simulink model "afe_rst_inv_psm_distributed_control_two_delays"  (R2026a)
settings: Solver=ode1be  StopTime=simlength  FixedStep=tc  MaxStep=Tc
values from neighbouring files (symbols this model uses):
  Amplitude_U = 1.16    [grid_fault_generator.m]
  Amplitude_V = Amplitude_U    (= 1.16)    [grid_fault_generator.m]
  Amplitude_W = Amplitude_U    (= 1.16)    [grid_fault_generator.m]
  end_time_LVRT = start_time_LVRT + error_length    [grid_fault_generator.m]
  Igrid_phase_normalization_factor = 270*sqrt(2)    [grid_emulator.m]
  omega_grid_emulator_nom = w_grid    (= 314.159265359)    [grid_emulator.m]
  omega_grid_nom = w_grid    (= 314.159265359)    [grid_emulator.m]
  t_ramp = 20e-3    (= 0.02)    [grid_fault_generator.m]
  ugrid_factor = 1    [grid_emulator.m]
  V_phase_normalization_factor = Vgrid_phase_normalization_factor    [grid_emulator.m]
  Vdc_bez = 1070    [grid_emulator.m]
  Vemu_ref_norm = Vemu_ref * sqrt(2) / V_phase_normalization_factor    [grid_emulator.m]
  vn_eta_pu = 0    [grid_emulator.m]
  vn_xi_pu = 0    [grid_emulator.m]
  vp_xi_pu = 1    [grid_emulator.m]
undefined symbols (not defined in the file or in its folder): Adrso, Aresd, Bresd, CFi, CFu, Cresd, Crso, CTRPIFF_CLIP_RELEASE, dead_time_INV, emf_fb_p, emf_fb_p_ccaller_1, emf_fb_p_ccaller_2, emf_p, emf_p_ccaller_1, emf_p_ccaller_2, fPWM_INV, g0_161Hz, g0_500Hz, g1_161Hz, g1_500Hz, i_grid_neg_eta_lim, i_grid_neg_eta_red_lim, i_grid_neg_xi_lim, i_grid_neg_xi_red_lim, i_grid_pos_eta_lim, i_grid_pos_eta_red_lim, ibez, id_lim, ieta_neg_ref_lim, ieta_pos_ref_lim, iq_lim, ixi_pos_ref_lim, Jm_norm, k_frt_ref, kg, ki_afe, ki_i, ki_id, ki_iq, ki_rc_neg_grid, ki_rc_pos_grid, ki_vs, ki_w, kp_afe, kp_i, kp_id, kp_iq, kp_rc_neg_grid, kp_rc_pos_grid, kp_vs, kp_w, kw, l1, l2, Lalpha_norm, Ld_norm, Ldrso, Lq_norm, Ls_norm, luenberger_l1 ... (+30)
libraries: fl_lib x146, nesl_utility x62, simulink x8, cstblocks_lti x7, sl_discontinuities x3, single_phase_transformer_lib x3, flexshaft_lib x1, permanent_magnet_synchronous_machine x1
(part 6 of 14)

== system afe_rst_inv_psm_distributed_control_two_delays/AFE-Modular/afe_leg_b/modulator/sv_pwm ==
  ab : Inport
  enable : Inport  Port=2
  Bus Selector : BusSelector  OutputSignals=da,db,dc
  Bus Selector1 : BusSelector  OutputSignals=us_alpha_ctrl,us_beta_ctrl
  C Caller : CCaller  FunctionName=sv_pwm_process_simulink  PortSpecificationStruct="%)30     .    N @   8    (     @         %    \"     4    !     0         %  0 \"0    $    _    07)G3F%M90  4&]R=$YA;64 4V-O<&4     26YD97@     5'EP90      4VEZ90      27-';&]B86P   X    P    !@    @    $          4    (     0    ,    !         !   P!O=70 #@   #     &    \"     0         !0    @    !     P    $         $  # &]U=  .    .     8    (    !          %    \"     $    &     0         0   ...(+2630 chars)"  SampleTime=ts_afe
  Constant : Constant  Value=ts_afe
  Data Type Conversion1 : DataTypeConversion  OutDataTypeStr=double  SaturateOnIntegerOverflow=off  RndMeth=Floor
  Data Type Conversion15 : DataTypeConversion  OutDataTypeStr=single  SaturateOnIntegerOverflow=off  RndMeth=Floor
  Data Type Conversion16 : DataTypeConversion  OutDataTypeStr=single  SaturateOnIntegerOverflow=off  RndMeth=Floor
  Data Type Conversion17 : DataTypeConversion  OutDataTypeStr=uint32  SaturateOnIntegerOverflow=off  RndMeth=Floor
  Data Type Conversion18 : DataTypeConversion  OutDataTypeStr=single  SaturateOnIntegerOverflow=off  RndMeth=Floor
  Data Type Conversion2 : DataTypeConversion  OutDataTypeStr=double  SaturateOnIntegerOverflow=off  RndMeth=Floor
  Data Type Conversion3 : DataTypeConversion  OutDataTypeStr=double  SaturateOnIntegerOverflow=off  RndMeth=Floor
  Zero-Order Hold{,1..3} (4 alike) : ZeroOrderHold  SampleTime=ts_afe
  modulator : Subsystem
  firing_gates : Outport
  wires:
  Bus Selector/3 -> Data Type Conversion3/1  "<dc>"
  Bus Selector/2 -> Data Type Conversion2/1  "<db>"
  Bus Selector/1 -> Data Type Conversion1/1  "<da>"
  Data Type Conversion1/1 -> modulator/1(u)  "du"
  Data Type Conversion2/1 -> modulator/2(v)  "dv"
  Data Type Conversion3/1 -> modulator/3(w)  "dw"
  Bus Selector1/2 -> Data Type Conversion15/1  "<us_beta_ctrl>"
  Bus Selector1/1 -> Data Type Conversion18/1  "<us_alpha_ctrl>"
  ab/1 -> Bus Selector1/1
  modulator/1(firing_gates) -> firing_gates/1
  C Caller/1 -> Bus Selector/1  "out"
  Data Type Conversion15/1 -> Zero-Order Hold1/1
  Zero-Order Hold3/1 -> C Caller/4
  Data Type Conversion17/1 -> Zero-Order Hold3/1
  Zero-Order Hold1/1 -> C Caller/2
  Data Type Conversion16/1 -> Zero-Order Hold2/1
  enable/1 -> Data Type Conversion17/1
  Data Type Conversion18/1 -> Zero-Order Hold/1
  Constant/1 -> Data Type Conversion16/1
  Zero-Order Hold2/1 -> C Caller/3
  Zero-Order Hold/1 -> C Caller/1

== system afe_rst_inv_psm_distributed_control_two_delays/AFE-Modular/afe_leg_b/solid_state_inverter/switch_1 ==
  Diode : fl_lib/Electrical/Electrical Elements/Diode  Vf=Vgamma V  Ron=Ron Ohm  Goff=1e-8 1/Ohm  i_specify=off  i_priority=None  i=0 A  i_nominal_specify=off  i_nominal_value=1  i_nominal_unit=A  v_specify=off  v_priority=None  v=0 V  v_nominal_specify=off  v_nominal_value=1  v_nominal_unit=V
  Switch : fl_lib/Electrical/Electrical Elements/Switch  R_closed=Ron Ohm  G_open=1e-8 1/Ohm  Threshold=7.5  i_specify=off  i_priority=None  i=0 A  i_nominal_specify=off  i_nominal_value=1  i_nominal_unit=A  v_specify=off  v_priority=None  v=0 V  v_nominal_specify=off  v_nominal_value=1  v_nominal_unit=V
  snubber : fl_lib/Electrical/Electrical Elements/Capacitor  c=Csnubber F  r=Rsnubber Ohm  g=0 1/Ohm  i_specify=off  i_priority=None  i=0 A  i_nominal_specify=off  i_nominal_value=1  i_nominal_unit=A  v_specify=off  v_priority=None  v=0 V  v_nominal_specify=off  v_nominal_value=1  v_nominal_unit=V  vc_specify=off  vc_priority=High  vc=0 V  vc_nominal_specify=off  vc_nominal_value=1  vc_nominal_unit=V
  G : PMIOPort  Side=Left
  C : PMIOPort  Port=2  Side=Left
  E : PMIOPort  Port=3  Side=Right
  connections:
  Diode/LConn1 -- snubber/RConn1 -- E/RConn1 -- Switch/LConn1
  Switch/RConn1 -- G/RConn1
  Diode/RConn1 -- snubber/LConn1 -- C/RConn1 -- Switch/RConn2

== system afe_rst_inv_psm_distributed_control_two_delays/AFE-Modular/afe_leg_b/solid_state_inverter/switch_2 ==
  Diode : fl_lib/Electrical/Electrical Elements/Diode  Vf=Vgamma V  Ron=Ron Ohm  Goff=1e-8 1/Ohm  i_specify=off  i_priority=None  i=0 A  i_nominal_specify=off  i_nominal_value=1  i_nominal_unit=A  v_specify=off  v_priority=None  v=0 V  v_nominal_specify=off  v_nominal_value=1  v_nominal_unit=V
  Switch : fl_lib/Electrical/Electrical Elements/Switch  R_closed=Ron Ohm  G_open=1e-8 1/Ohm  Threshold=7.5  i_specify=off  i_priority=None  i=0 A  i_nominal_specify=off  i_nominal_value=1  i_nominal_unit=A  v_specify=off  v_priority=None  v=0 V  v_nominal_specify=off  v_nominal_value=1  v_nominal_unit=V
  snubber : fl_lib/Electrical/Electrical Elements/Capacitor  c=Csnubber F  r=Rsnubber Ohm  g=0 1/Ohm  i_specify=off  i_priority=None  i=0 A  i_nominal_specify=off  i_nominal_value=1  i_nominal_unit=A  v_specify=off  v_priority=None  v=0 V  v_nominal_specify=off  v_nominal_value=1  v_nominal_unit=V  vc_specify=off  vc_priority=High  vc=0 V  vc_nominal_specify=off  vc_nominal_value=1  vc_nominal_unit=V
  G : PMIOPort  Side=Left
  C : PMIOPort  Port=2  Side=Left
  E : PMIOPort  Port=3  Side=Right
  connections:
  Diode/RConn1 -- snubber/LConn1 -- Switch/RConn2 -- C/RConn1
  Switch/RConn1 -- G/RConn1
  Diode/LConn1 -- snubber/RConn1 -- Switch/LConn1 -- E/RConn1

== system afe_rst_inv_psm_distributed_control_two_delays/AFE-Modular/afe_leg_c/driver_board_c/current_ctrl ==
  i_xi_ref : Inport
  phase_current_control : Subsystem
  xieta2abc : Subsystem
  us_alphabeta_ctrl : Outport
  wires:
  i_xi_ref/1 -> xieta2abc/1(pos_xi)  "i_xi_ref"
  phase_current_control/1(us_alphabeta_ctrl) -> us_alphabeta_ctrl/1
  xieta2abc/1(i_abc_reference) -> phase_current_control/1(In1)
  [gamma_grid_dbc] -> xieta2abc/5(gamma)
  [isc_pu_dbc] -> phase_current_control/2(is_abc)
  [is_eta_pos_ref_mb_fb_dbc] -> xieta2abc/2(pos_eta)
  [is_xi_neg_ref_mb_fb_dbc] -> xieta2abc/3(neg_xi)
  [is_eta_neg_ref_mb_fb_dbc] -> xieta2abc/4(neg_eta)

== system afe_rst_inv_psm_distributed_control_two_delays/AFE-Modular/afe_leg_c/driver_board_c/dq_pll ==
  pll_stageA : Subsystem
  pll_stageB : Subsystem
  tag scope: gamma_grid_dbc=global
  wires:
  pll_stageB/1(gamma_grid_pll) -> pll_stageA/1(gamma_grid), [gamma_grid_dbc]
  pll_stageA/2(u_grid_pos_eta) -> pll_stageB/2(u_grid_pos_eta)  "u_grid_pos_eta"
  pll_stageA/1(u_grid_pos_xi) -> pll_stageB/1(u_grid_pos_xi)  "u_grid_pos_xi"

== system afe_rst_inv_psm_distributed_control_two_delays/AFE-Modular/afe_leg_c/driver_board_c/igc_dbc_estimator ==
  Gain : Gain  Gain=omega_grid_nom*CFu
  Sum : Sum  Inputs=|++
  quadrature_shift_filter : MATLAB Function  TreatAsAtomicUnit=on  SystemSampleTime=ts_afe
  tag scope: igc_pu_dbc=global
  wires:
  Sum/1 -> [igc_pu_dbc]
  quadrature_shift_filter/1(y) -> Sum/2
  [ugc_pu_dbc] -> Gain/1
  [isc_pu_dbc] -> Sum/1
  Gain/1 -> quadrature_shift_filter/1(input)

== system afe_rst_inv_psm_distributed_control_two_delays/AFE-Modular/afe_leg_c/driver_board_c/voltage-current-acquisition ==
  is_eta_neg_ref_fieldbus : Subsystem
  is_eta_pos_ref_fieldbus : Subsystem
  is_xi_neg_ref_fieldbus : Subsystem
  isb_fieldbus : Subsystem
  isc_fieldbus : Subsystem
  isc_measure_and_normalization : Subsystem
  ixi_ref_fieldbus : Subsystem
  ixi_ref_fieldbus1 : Subsystem
  ub_ctrl_fieldbus : Subsystem
  uc_ctrl_fieldbus : Subsystem
  uga_fieldbus : Subsystem
  ugb_fieldbus : Subsystem
  ugc_measure_and_normalization : Subsystem
  tag scope: is_eta_neg_ref_mb_fb_dbc=global, is_eta_pos_ref_mb_fb_dbc=global, is_xi_neg_ref_mb_fb_dbc=global, isa_pu_dba_fb_dbc=global, isb_pu_dbb_fb_dbc=global, isc_pu_dbc=global, ixi_ref_dba_fb_dbc=global, ixi_ref_dbb_fb_dbc=global, uga_pu_dba_fb_dbc=global, ugb_pu_dbb_fb_dbc=global, ugc_pu_dbc=global, usa_ctrl_dba_fb_dbc=global, usb_ctrl_dbb_fb_dbc=global
  wires:
  ub_ctrl_fieldbus/1(u_ctrl_fb) -> [usa_ctrl_dba_fb_dbc]
  [isb_pu_dbb] -> isc_fieldbus/1(is)
  isb_fieldbus/1(is_fb) -> [isa_pu_dba_fb_dbc]
  [usb_ctrl_dbb] -> uc_ctrl_fieldbus/1(u_ctrl)
  isc_measure_and_normalization/1(is_pu) -> [isc_pu_dbc]
  [isa_pu_dba] -> isb_fieldbus/1(is)
  [usa_ctrl_dba] -> ub_ctrl_fieldbus/1(u_ctrl)
  [isc_dbc] -> isc_measure_and_normalization/1(is)
  uc_ctrl_fieldbus/1(u_ctrl_fb) -> [usb_ctrl_dbb_fb_dbc]
  isc_fieldbus/1(is_fb) -> [isb_pu_dbb_fb_dbc]
  [ugc_dbc] -> ugc_measure_and_normalization/1(ug)
  ugc_measure_and_normalization/1(ug_pu) -> [ugc_pu_dbc]
  [ugb_pu_dbb] -> ugb_fieldbus/1(ug)
  [uga_pu_dba] -> uga_fieldbus/1(ug)
  ugb_fieldbus/1(ug_fb) -> [ugb_pu_dbb_fb_dbc]
  uga_fieldbus/1(ug_fb) -> [uga_pu_dba_fb_dbc]
  ixi_ref_fieldbus/1(is_fb) -> [ixi_ref_dba_fb_dbc]
  ixi_ref_fieldbus1/1(is_fb) -> [ixi_ref_dbb_fb_dbc]
  [ixi_ref_dbb] -> ixi_ref_fieldbus1/1(is)
  [ixi_ref_dba] -> ixi_ref_fieldbus/1(is)
  [i_stack_pos_eta_ref] -> is_eta_pos_ref_fieldbus/1(is)
  [i_stack_neg_eta_ref] -> is_eta_neg_ref_fieldbus/1(is)
  [i_stack_neg_xi_ref] -> is_xi_neg_ref_fieldbus/1(is)
  is_eta_pos_ref_fieldbus/1(is_fb) -> [is_eta_pos_ref_mb_fb_dbc]
  is_eta_neg_ref_fieldbus/1(is_fb) -> [is_eta_neg_ref_mb_fb_dbc]
  is_xi_neg_ref_fieldbus/1(is_fb) -> [is_xi_neg_ref_mb_fb_dbc]

== system afe_rst_inv_psm_distributed_control_two_delays/AFE-Modular/afe_leg_c/modulator/sv_pwm ==
  u_alphabeta_ctrl : Inport
  enable : Inport  Port=2
  Bus Selector : BusSelector  OutputSignals=da,db,dc
  Bus Selector1 : BusSelector  OutputSignals=us_alpha_ctrl,us_beta_ctrl
  C Caller : CCaller  FunctionName=sv_pwm_process_simulink  PortSpecificationStruct="%)30     .    N @   8    (     @         %    \"     4    !     0         %  0 \"0    $    _    07)G3F%M90  4&]R=$YA;64 4V-O<&4     26YD97@     5'EP90      4VEZ90      27-';&]B86P   X    P    !@    @    $          4    (     0    ,    !         !   P!O=70 #@   #     &    \"     0         !0    @    !     P    $         $  # &]U=  .    .     8    (    !          %    \"     $    &     0         0   ...(+2630 chars)"  SampleTime=ts_afe
  Constant : Constant  Value=ts_afe
  Data Type Conversion1 : DataTypeConversion  OutDataTypeStr=double  SaturateOnIntegerOverflow=off  RndMeth=Floor
  Data Type Conversion15 : DataTypeConversion  OutDataTypeStr=single  SaturateOnIntegerOverflow=off  RndMeth=Floor
  Data Type Conversion16 : DataTypeConversion  OutDataTypeStr=single  SaturateOnIntegerOverflow=off  RndMeth=Floor
  Data Type Conversion17 : DataTypeConversion  OutDataTypeStr=uint32  SaturateOnIntegerOverflow=off  RndMeth=Floor
  Data Type Conversion18 : DataTypeConversion  OutDataTypeStr=single  SaturateOnIntegerOverflow=off  RndMeth=Floor
  Data Type Conversion2 : DataTypeConversion  OutDataTypeStr=double  SaturateOnIntegerOverflow=off  RndMeth=Floor
  Data Type Conversion3 : DataTypeConversion  OutDataTypeStr=double  SaturateOnIntegerOverflow=off  RndMeth=Floor
  Zero-Order Hold{,1..3} (4 alike) : ZeroOrderHold  SampleTime=ts_afe
  modulator : Subsystem
  firing_gates : Outport
  wires:
  Zero-Order Hold/1 -> C Caller/1
  Zero-Order Hold2/1 -> C Caller/3
  Constant/1 -> Data Type Conversion16/1
  Data Type Conversion18/1 -> Zero-Order Hold/1
  enable/1 -> Data Type Conversion17/1
  Data Type Conversion16/1 -> Zero-Order Hold2/1
  Zero-Order Hold1/1 -> C Caller/2
  Data Type Conversion17/1 -> Zero-Order Hold3/1
  Zero-Order Hold3/1 -> C Caller/4
  Data Type Conversion15/1 -> Zero-Order Hold1/1
  C Caller/1 -> Bus Selector/1  "out"
  modulator/1(firing_gates) -> firing_gates/1
  u_alphabeta_ctrl/1 -> Bus Selector1/1
  Bus Selector1/1 -> Data Type Conversion18/1  "<us_alpha_ctrl>"
  Bus Selector1/2 -> Data Type Conversion15/1  "<us_beta_ctrl>"
  Data Type Conversion3/1 -> modulator/3(w)  "dw"
  Data Type Conversion2/1 -> modulator/2(v)  "dv"
  Data Type Conversion1/1 -> modulator/1(u)  "du"
  Bus Selector/1 -> Data Type Conversion1/1  "<da>"
  Bus Selector/2 -> Data Type Conversion2/1  "<db>"
  Bus Selector/3 -> Data Type Conversion3/1  "<dc>"

== system afe_rst_inv_psm_distributed_control_two_delays/AFE-Modular/afe_leg_c/solid_state_inverter/switch_1 ==
  Diode : fl_lib/Electrical/Electrical Elements/Diode  Vf=Vgamma V  Ron=Ron Ohm  Goff=1e-8 1/Ohm  i_specify=off  i_priority=None  i=0 A  i_nominal_specify=off  i_nominal_value=1  i_nominal_unit=A  v_specify=off  v_priority=None  v=0 V  v_nominal_specify=off  v_nominal_value=1  v_nominal_unit=V
  Switch : fl_lib/Electrical/Electrical Elements/Switch  R_closed=Ron Ohm  G_open=1e-8 1/Ohm  Threshold=7.5  i_specify=off  i_priority=None  i=0 A  i_nominal_specify=off  i_nominal_value=1  i_nominal_unit=A  v_specify=off  v_priority=None  v=0 V  v_nominal_specify=off  v_nominal_value=1  v_nominal_unit=V
  snubber : fl_lib/Electrical/Electrical Elements/Capacitor  c=Csnubber F  r=Rsnubber Ohm  g=0 1/Ohm  i_specify=off  i_priority=None  i=0 A  i_nominal_specify=off  i_nominal_value=1  i_nominal_unit=A  v_specify=off  v_priority=None  v=0 V  v_nominal_specify=off  v_nominal_value=1  v_nominal_unit=V  vc_specify=off  vc_priority=High  vc=0 V  vc_nominal_specify=off  vc_nominal_value=1  vc_nominal_unit=V
  G : PMIOPort  Side=Left
  C : PMIOPort  Port=2  Side=Left
  E : PMIOPort  Port=3  Side=Right
  connections:
  Switch/RConn2 -- C/RConn1 -- snubber/LConn1 -- Diode/RConn1
  Switch/RConn1 -- G/RConn1
  Switch/LConn1 -- E/RConn1 -- snubber/RConn1 -- Diode/LConn1

== system afe_rst_inv_psm_distributed_control_two_delays/AFE-Modular/afe_leg_c/solid_state_inverter/switch_2 ==
  Diode : fl_lib/Electrical/Electrical Elements/Diode  Vf=Vgamma V  Ron=Ron Ohm  Goff=1e-8 1/Ohm  i_specify=off  i_priority=None  i=0 A  i_nominal_specify=off  i_nominal_value=1  i_nominal_unit=A  v_specify=off  v_priority=None  v=0 V  v_nominal_specify=off  v_nominal_value=1  v_nominal_unit=V
  Switch : fl_lib/Electrical/Electrical Elements/Switch  R_closed=Ron Ohm  G_open=1e-8 1/Ohm  Threshold=7.5  i_specify=off  i_priority=None  i=0 A  i_nominal_specify=off  i_nominal_value=1  i_nominal_unit=A  v_specify=off  v_priority=None  v=0 V  v_nominal_specify=off  v_nominal_value=1  v_nominal_unit=V
  snubber : fl_lib/Electrical/Electrical Elements/Capacitor  c=Csnubber F  r=Rsnubber Ohm  g=0 1/Ohm  i_specify=off  i_priority=None  i=0 A  i_nominal_specify=off  i_nominal_value=1  i_nominal_unit=A  v_specify=off  v_priority=None  v=0 V  v_nominal_specify=off  v_nominal_value=1  v_nominal_unit=V  vc_specify=off  vc_priority=High  vc=0 V  vc_nominal_specify=off  vc_nominal_value=1  vc_nominal_unit=V
  G : PMIOPort  Side=Left
  C : PMIOPort  Port=2  Side=Left
  E : PMIOPort  Port=3  Side=Right
  connections:
  E/RConn1 -- Switch/LConn1 -- snubber/RConn1 -- Diode/LConn1
  Switch/RConn1 -- G/RConn1
  C/RConn1 -- Switch/RConn2 -- snubber/LConn1 -- Diode/RConn1

== system afe_rst_inv_psm_distributed_control_two_delays/INV-Modular/inv_leg_u/driver_board_u/double_integrator_observer ==
  theta : Inport
  Gain : Gain  Gain=kw
  Gain1 : Gain  Gain=kg
  Gain4 : Gain  Gain=omega_bez
  Gain5 : Gain  Gain=ts_inv
  Gain6 : Gain  Gain=1/omega_bez
  Sum : Sum  Inputs=-+|
  Sum1 : Sum  Inputs=|++
  Sum2 : Sum  Inputs=|++
  Sum8 : Sum  Inputs=++|
  Unit Delay1 : UnitDelay  SampleTime=ts_inv
  Unit Delay2 : UnitDelay  SampleTime=ts_inv
  bounder1 : MATLAB Function  TreatAsAtomicUnit=on  SystemSampleTime=ts_inv
  bounder2 : MATLAB Function  TreatAsAtomicUnit=on  SystemSampleTime=ts_inv
  omega_pu_hat : Outport  VectorParamsAs1DForOutWhenUnconnected=off
  theta_hat : Outport  Port=2  VectorParamsAs1DForOutWhenUnconnected=off
  wires:
  theta/1 -> Sum/2  "theta"
  Sum8/1 -> bounder2/1(u)
  Sum1/1 -> Unit Delay2/1
  Unit Delay2/1 -> omega_pu_hat/1, Sum1/2, Gain5/1
  Sum2/1 -> Sum8/2
  bounder2/1(y) -> Unit Delay1/1
  bounder1/1(y) -> Gain/1, Gain1/1
  Gain5/1 -> Gain4/1
  Sum/1 -> bounder1/1(u)
  Unit Delay1/1 -> Sum2/2, theta_hat/1, Sum/1  "theta_hat"
  Gain/1 -> Gain6/1
  Gain6/1 -> Sum1/1
  Gain4/1 -> Sum8/1
  Gain1/1 -> Sum2/1

== system afe_rst_inv_psm_distributed_control_two_delays/INV-Modular/inv_leg_u/driver_board_u/motor_vector_control ==
  motor_torque_ref : Inport
  Bus Creator1 : BusCreator  Inputs=2
  Unit Delay2 : UnitDelay  SampleTime=ts_inv
  Unit Delay3 : UnitDelay  SampleTime=ts_inv
  Variant Source : VariantSource  VariantControls={use_psm_encoder == 1, use_psm_encoder == 0}
  bemf_observer : Subsystem
  current_ctrl : Subsystem
  current_transformation : Subsystem
  dq2alphabeta : MATLAB Function  TreatAsAtomicUnit=on  SystemSampleTime=ts_inv
  us_alphabeta_ctrl : Outport
  tag scope: motor_ualpha_ctrl_dbu=global, motor_ubeta_ctrl_dbu=global
  wires:
  Unit Delay3/1 -> [motor_ubeta_ctrl_dbu]
  dq2alphabeta/1(alpha) -> Unit Delay2/1
  Variant Source/1 -> current_transformation/4(gamma), dq2alphabeta/3(gamma)
  [isw_pu_dbw_fb_dbu] -> current_transformation/3(w)
  Unit Delay2/1 -> [motor_ualpha_ctrl_dbu]
  current_ctrl/2(uq) -> dq2alphabeta/2(q)
  current_ctrl/1(ud) -> dq2alphabeta/1(d)
  [motor_ialpha_pu_dbu] -> bemf_observer/1(ialpha_pu)
  [motor_ubeta_ctrl_dbu] -> bemf_observer/4(ubeta_pu)
  [motor_ualpha_ctrl_dbu] -> bemf_observer/3(ualpha_pu)
  [motor_ualpha_ctrl_dbu] -> Bus Creator1/1  "motor_ualpha_ctrl"
  [isu_pu_dbu] -> current_transformation/1(u)
  [motor_ubeta_ctrl_dbu] -> Bus Creator1/2  "motor_ubeta_ctrl"
  [motor_ibeta_pu_dbu] -> bemf_observer/2(ibeta_pu)
  dq2alphabeta/2(beta) -> Unit Delay3/1
  motor_torque_ref/1 -> current_ctrl/1(iq_ref)  "motor_torque_ref"
  Bus Creator1/1 -> us_alphabeta_ctrl/1
  [isv_pu_dbv_fb_dbu] -> current_transformation/2(v)
  [motor_theta_hat_dbu] -> Variant Source/2
  [motor_phase_mb_fb_dbu_luenberger] -> Variant Source/1

== system afe_rst_inv_psm_distributed_control_two_delays/INV-Modular/inv_leg_u/driver_board_u/psm_speed_ctrl ==
  motor_omega : Inport
  motor_omega_ref : Inport  Port=2
  1/Ti : Gain  Gain=kp_w  SaturateOnIntegerOverflow=on  OutDataTypeStr=Inherit: Same as input  ParamDataTypeStr=Inherit: Same as input
  Sum1 : Sum  Inputs=+++  SaturateOnIntegerOverflow=on
  Sum2 : Sum  Inputs=-+  SaturateOnIntegerOverflow=on
  Sum3 : Sum  Inputs=-+  SaturateOnIntegerOverflow=on
  Unit Delay4 : UnitDelay  SampleTime=ts_inv
  iq_lim : Saturate  UpperLimit=iq_lim  LowerLimit=-iq_lim
  kp : Gain  Gain=ki_w*ts_inv  SaturateOnIntegerOverflow=on  OutDataTypeStr=Inherit: Same as input  ParamDataTypeStr=Inherit: Same as input
  motor_torque_ref : Outport
  wires:
  iq_lim/1 -> motor_torque_ref/1, Sum3/2
  Sum1/1 -> iq_lim/1
  Sum2/1 -> 1/Ti/1, kp/1
  motor_omega/1 -> Sum2/1
  motor_omega_ref/1 -> Sum2/2
  Unit Delay4/1 -> Sum1/3
  Sum3/1 -> Unit Delay4/1
  kp/1 -> Sum1/2
  1/Ti/1 -> Sum3/1, Sum1/1

== system afe_rst_inv_psm_distributed_control_two_delays/INV-Modular/inv_leg_u/driver_board_u/torque_curve ==
  rotor speed : Inport
  1-D Lookup Table : Lookup_n-D  NumberOfTableDimensions=1  BreakpointsForDimension1Source=Input port  BreakpointsForDimension1=[-5:5]  TableSource=Input port  Table=tanh([-5:5])  InterpMethod=Linear Lagrange  InternalRulePriority=Speed  RndMeth=Simplest
      settings: InputPortMap=u0,p221,p5
  Constant : Constant  Value=rpm_base'
  Constant1 : Constant  Value=torque_base'
  Gain : Gain  Gain=-1
  Gain1 : Gain  Gain=pp/60*2*pi/omega_bez
  Gain2 : Gain  Gain=1e3/tau_bez
  Saturation : Saturate  UpperLimit=0  LowerLimit=-inf
  omega_hat_flt : Subsystem
  torque_ref : Outport
  wires:
  rotor speed/1 -> omega_hat_flt/1(omega_hat)
  Gain2/1 -> 1-D Lookup Table/2
  1-D Lookup Table/1 -> Gain/1
  Constant/1 -> Gain1/1
  Constant1/1 -> Gain2/1
  Gain1/1 -> 1-D Lookup Table/3
  Gain/1 -> Saturation/1
  Saturation/1 -> torque_ref/1
  omega_hat_flt/1(omega_hat_flt) -> 1-D Lookup Table/1

== system afe_rst_inv_psm_distributed_control_two_delays/INV-Modular/inv_leg_u/driver_board_u/voltage-current-acquisition ==
  From4 : From  Commented=on  GotoTag=usv_ctrl_dbv  TagVisibility=global
  From7 : From  Commented=on  GotoTag=usw_ctrl_dbw  TagVisibility=global
  Goto7 : Goto  Commented=on  GotoTag=usv_ctrl_dbv_fb_dbu  TagVisibility=global
  Goto8 : Goto  Commented=on  GotoTag=usw_ctrl_dbw_fb_dbu  TagVisibility=global
  isu_measure : Subsystem
  isv_fieldbus : Subsystem
  isw_fieldbus : Subsystem
  motor_phase_fieldbus : Subsystem
  usu_measure : Subsystem
  usv_ctrl_fieldbus : Subsystem  Commented=on
  usv_fieldbus : Subsystem
  usw_ctrl_fieldbus : Subsystem  Commented=on
  usw_fieldbus : Subsystem
  tag scope: isu_pu_dbu=global, isv_pu_dbv_fb_dbu=global, isw_pu_dbw_fb_dbu=global, motor_phase_mb_fb_dbu=global, usu_pu_dbu=global, usv_pu_dbv_fb_dbu=global, usw_pu_dbw_fb_dbu=global
  wires:
  usv_fieldbus/1(us_fb) -> [usv_pu_dbv_fb_dbu]
  usw_fieldbus/1(us_fb) -> [usw_pu_dbw_fb_dbu]
  [usv_pu_dbv] -> usv_fieldbus/1(us)
  [usw_pu_dbw] -> usw_fieldbus/1(us)
  usu_measure/1(us_pu) -> [usu_pu_dbu]
  [usu_dbu] -> usu_measure/1(us)
  isw_fieldbus/1(is_fb) -> [isw_pu_dbw_fb_dbu]
  [isu_dbu] -> isu_measure/1(is)
  [isv_pu_dbv] -> isv_fieldbus/1(is)
  isu_measure/1(is_pu) -> [isu_pu_dbu]
  isv_fieldbus/1(is_fb) -> [isv_pu_dbv_fb_dbu]
  [isw_pu_dbw] -> isw_fieldbus/1(is)
  [motor_phase_mb] -> motor_phase_fieldbus/1(motor_phase)
  motor_phase_fieldbus/1(motor_phase_fb) -> [motor_phase_mb_fb_dbu]
  usv_ctrl_fieldbus/1(u_ctrl_fb) -> Goto7/1
  usw_ctrl_fieldbus/1(u_ctrl_fb) -> Goto8/1
  From7/1 -> usw_ctrl_fieldbus/1(u_ctrl)
  From4/1 -> usv_ctrl_fieldbus/1(u_ctrl)

== system afe_rst_inv_psm_distributed_control_two_delays/INV-Modular/inv_leg_u/modulator/sv_pwm ==
  ab : Inport
  enable : Inport  Port=2
  Bus Selector : BusSelector  OutputSignals=da
  Bus Selector1 : BusSelector  OutputSignals=motor_ualpha_ctrl,motor_ubeta_ctrl
  C Caller : CCaller  FunctionName=sv_pwm_process_simulink  PortSpecificationStruct="%)30     .    N @   8    (     @         %    \"     4    !     0         %  0 \"0    $    _    07)G3F%M90  4&]R=$YA;64 4V-O<&4     26YD97@     5'EP90      4VEZ90      27-';&]B86P   X    P    !@    @    $          4    (     0    ,    !         !   P!O=70 #@   #     &    \"     0         !0    @    !     P    $         $  # &]U=  .    .     8    (    !          %    \"     $    &     0         0   ...(+2630 chars)"  SampleTime=ts_inv
  Constant : Constant  Value=ts_inv
  Data Type Conversion1 : DataTypeConversion  OutDataTypeStr=double  SaturateOnIntegerOverflow=off  RndMeth=Floor
  Data Type Conversion15 : DataTypeConversion  OutDataTypeStr=single  SaturateOnIntegerOverflow=off  RndMeth=Floor
  Data Type Conversion16 : DataTypeConversion  OutDataTypeStr=single  SaturateOnIntegerOverflow=off  RndMeth=Floor
  Data Type Conversion17 : DataTypeConversion  OutDataTypeStr=uint32  SaturateOnIntegerOverflow=off  RndMeth=Floor
  Data Type Conversion18 : DataTypeConversion  OutDataTypeStr=single  SaturateOnIntegerOverflow=off  RndMeth=Floor
  Zero-Order Hold{,1..3} (4 alike) : ZeroOrderHold  SampleTime=ts_afe
  alphabeta2uvw : MATLAB Function  TreatAsAtomicUnit=on  SystemSampleTime=ts_afe
  modulator : Subsystem
  firing_gates : Outport
  tag scope: inv_mu=global, inv_mv=global, inv_mw=global
  wires:
  alphabeta2uvw/3(w) -> [inv_mw]  "mw"
  alphabeta2uvw/1(u) -> [inv_mu]  "mu"
  alphabeta2uvw/2(v) -> [inv_mv]  "mv"
  Data Type Conversion1/1 -> modulator/1(u)  "du"
  Bus Selector1/2 -> Data Type Conversion15/1, alphabeta2uvw/2(beta)  "<motor_ubeta_ctrl>"
  Bus Selector1/1 -> Data Type Conversion18/1, alphabeta2uvw/1(alpha)  "<motor_ualpha_ctrl>"
  ab/1 -> Bus Selector1/1
  modulator/1(firing_gates) -> firing_gates/1
  C Caller/1 -> Bus Selector/1  "out"
  Data Type Conversion15/1 -> Zero-Order Hold1/1
  Zero-Order Hold3/1 -> C Caller/4
  Data Type Conversion17/1 -> Zero-Order Hold3/1
  Zero-Order Hold1/1 -> C Caller/2
  Data Type Conversion16/1 -> Zero-Order Hold2/1
  enable/1 -> Data Type Conversion17/1
  Data Type Conversion18/1 -> Zero-Order Hold/1
  Constant/1 -> Data Type Conversion16/1
  Zero-Order Hold2/1 -> C Caller/3
  Zero-Order Hold/1 -> C Caller/1
  Bus Selector/1 -> Data Type Conversion1/1  "<da>"

== system afe_rst_inv_psm_distributed_control_two_delays/INV-Modular/inv_leg_u/solid_state_inverter/switch_1 ==
  Diode : fl_lib/Electrical/Electrical Elements/Diode  Vf=Vgamma V  Ron=Ron Ohm  Goff=1e-8 1/Ohm  i_specify=off  i_priority=None  i=0 A  i_nominal_specify=off  i_nominal_value=1  i_nominal_unit=A  v_specify=off  v_priority=None  v=0 V  v_nominal_specify=off  v_nominal_value=1  v_nominal_unit=V
  Switch : fl_lib/Electrical/Electrical Elements/Switch  R_closed=Ron Ohm  G_open=1e-8 1/Ohm  Threshold=7.5  i_specify=off  i_priority=None  i=0 A  i_nominal_specify=off  i_nominal_value=1  i_nominal_unit=A  v_specify=off  v_priority=None  v=0 V  v_nominal_specify=off  v_nominal_value=1  v_nominal_unit=V
  snubber : fl_lib/Electrical/Electrical Elements/Capacitor  c=Csnubber F  r=Rsnubber Ohm  g=0 1/Ohm  i_specify=off  i_priority=None  i=0 A  i_nominal_specify=off  i_nominal_value=1  i_nominal_unit=A  v_specify=off  v_priority=None  v=0 V  v_nominal_specify=off  v_nominal_value=1  v_nominal_unit=V  vc_specify=off  vc_priority=High  vc=0 V  vc_nominal_specify=off  vc_nominal_value=1  vc_nominal_unit=V
  G : PMIOPort  Side=Left
  C : PMIOPort  Port=2  Side=Left
  E : PMIOPort  Port=3  Side=Right
  connections:
  Diode/LConn1 -- snubber/RConn1 -- E/RConn1 -- Switch/LConn1
  Switch/RConn1 -- G/RConn1
  Diode/RConn1 -- snubber/LConn1 -- C/RConn1 -- Switch/RConn2

== system afe_rst_inv_psm_distributed_control_two_delays/INV-Modular/inv_leg_u/solid_state_inverter/switch_2 ==
  Diode : fl_lib/Electrical/Electrical Elements/Diode  Vf=Vgamma V  Ron=Ron Ohm  Goff=1e-8 1/Ohm  i_specify=off  i_priority=None  i=0 A  i_nominal_specify=off  i_nominal_value=1  i_nominal_unit=A  v_specify=off  v_priority=None  v=0 V  v_nominal_specify=off  v_nominal_value=1  v_nominal_unit=V
  Switch : fl_lib/Electrical/Electrical Elements/Switch  R_closed=Ron Ohm  G_open=1e-8 1/Ohm  Threshold=7.5  i_specify=off  i_priority=None  i=0 A  i_nominal_specify=off  i_nominal_value=1  i_nominal_unit=A  v_specify=off  v_priority=None  v=0 V  v_nominal_specify=off  v_nominal_value=1  v_nominal_unit=V
  snubber : fl_lib/Electrical/Electrical Elements/Capacitor  c=Csnubber F  r=Rsnubber Ohm  g=0 1/Ohm  i_specify=off  i_priority=None  i=0 A  i_nominal_specify=off  i_nominal_value=1  i_nominal_unit=A  v_specify=off  v_priority=None  v=0 V  v_nominal_specify=off  v_nominal_value=1  v_nominal_unit=V  vc_specify=off  vc_priority=High  vc=0 V  vc_nominal_specify=off  vc_nominal_value=1  vc_nominal_unit=V
  G : PMIOPort  Side=Left
  C : PMIOPort  Port=2  Side=Left
  E : PMIOPort  Port=3  Side=Right
  connections:
  Diode/RConn1 -- snubber/LConn1 -- Switch/RConn2 -- C/RConn1
  Switch/RConn1 -- G/RConn1
  Diode/LConn1 -- snubber/RConn1 -- Switch/LConn1 -- E/RConn1

== system afe_rst_inv_psm_distributed_control_two_delays/INV-Modular/inv_leg_v/driver_board_v/double_integrator_observer ==
  theta : Inport
  Gain : Gain  Gain=kw
  Gain1 : Gain  Gain=kg
  Gain4 : Gain  Gain=omega_bez
  Gain5 : Gain  Gain=ts_inv
  Gain6 : Gain  Gain=1/omega_bez
  Sum : Sum  Inputs=-+|
  Sum1 : Sum  Inputs=|++
  Sum2 : Sum  Inputs=|++
  Sum8 : Sum  Inputs=++|
  Unit Delay1 : UnitDelay  SampleTime=ts_inv
  Unit Delay2 : UnitDelay  SampleTime=ts_inv
  bounder1 : MATLAB Function  TreatAsAtomicUnit=on  SystemSampleTime=ts_inv
  bounder2 : MATLAB Function  TreatAsAtomicUnit=on  SystemSampleTime=ts_inv
  omega_pu_hat : Outport  VectorParamsAs1DForOutWhenUnconnected=off
  theta_hat : Outport  Port=2  VectorParamsAs1DForOutWhenUnconnected=off
  wires:
  theta/1 -> Sum/2  "theta"
  Sum8/1 -> bounder2/1(u)
  Sum1/1 -> Unit Delay2/1
  Unit Delay2/1 -> omega_pu_hat/1, Sum1/2, Gain5/1
  Sum2/1 -> Sum8/2
  bounder2/1(y) -> Unit Delay1/1
  bounder1/1(y) -> Gain/1, Gain1/1
  Gain5/1 -> Gain4/1
  Sum/1 -> bounder1/1(u)
  Unit Delay1/1 -> Sum2/2, theta_hat/1, Sum/1  "theta_hat"
  Gain/1 -> Gain6/1
  Gain6/1 -> Sum1/1
  Gain4/1 -> Sum8/1
  Gain1/1 -> Sum2/1

== system afe_rst_inv_psm_distributed_control_two_delays/INV-Modular/inv_leg_v/driver_board_v/motor_vector_control ==
  motor_torque_ref : Inport
  Bus Creator1 : BusCreator  Inputs=2
  Unit Delay2 : UnitDelay  SampleTime=ts_inv
  Unit Delay3 : UnitDelay  SampleTime=ts_inv
  Variant Source : VariantSource  VariantControls={use_psm_encoder == 1, use_psm_encoder == 0}
  bemf_observer : Subsystem
  current_ctrl : Subsystem
  current_transformation : Subsystem
  dq2alphabeta : MATLAB Function  TreatAsAtomicUnit=on  SystemSampleTime=ts_inv
  us_alphabeta_ctrl : Outport
  tag scope: motor_ualpha_ctrl_dbv=global, motor_ubeta_ctrl_dbv=global
  wires:
  [isv_pu_dbv] -> current_transformation/2(v)
  Bus Creator1/1 -> us_alphabeta_ctrl/1
  motor_torque_ref/1 -> current_ctrl/1(iq_ref)  "motor_torque_ref"
  dq2alphabeta/2(beta) -> Unit Delay3/1
  [motor_ibeta_pu_dbv] -> bemf_observer/2(ibeta_pu)
  [motor_ubeta_ctrl_dbv] -> Bus Creator1/2  "motor_ubeta_ctrl"
  [isu_pu_dbu_fb_dbv] -> current_transformation/1(u)
  [motor_ualpha_ctrl_dbv] -> Bus Creator1/1  "motor_ualpha_ctrl"
  [motor_ualpha_ctrl_dbv] -> bemf_observer/3(ualpha_pu)
  [motor_ubeta_ctrl_dbv] -> bemf_observer/4(ubeta_pu)
  [motor_ialpha_pu_dbv] -> bemf_observer/1(ialpha_pu)
  current_ctrl/1(ud) -> dq2alphabeta/1(d)
  current_ctrl/2(uq) -> dq2alphabeta/2(q)
  Unit Delay2/1 -> [motor_ualpha_ctrl_dbv]
  [isw_pu_dbw_fb_dbv] -> current_transformation/3(w)
  Variant Source/1 -> current_transformation/4(gamma), dq2alphabeta/3(gamma)
  dq2alphabeta/1(alpha) -> Unit Delay2/1
  Unit Delay3/1 -> [motor_ubeta_ctrl_dbv]
  [motor_theta_hat_dbv] -> Variant Source/2
  [motor_phase_mb_fb_dbv_luenberger] -> Variant Source/1

== system afe_rst_inv_psm_distributed_control_two_delays/INV-Modular/inv_leg_v/driver_board_v/voltage-current-acquisition ==
  From7 : From  Commented=on  GotoTag=usu_ctrl_dbu  TagVisibility=global
  From8 : From  Commented=on  GotoTag=usw_ctrl_dbw  TagVisibility=global
  Goto8 : Goto  Commented=on  GotoTag=usu_ctrl_dbu_fb_dbv  TagVisibility=global
  Goto9 : Goto  Commented=on  GotoTag=usw_ctrl_dbw_fb_dbw  TagVisibility=global
  isu_measure : Subsystem
  isv_fieldbus : Subsystem
  isw_fieldbus : Subsystem
  motor_phase_fieldbus : Subsystem
  motor_torque_fieldbus : Subsystem
  usu_ctrl_fieldbus : Subsystem  Commented=on
  usu_fieldbus : Subsystem
  usv_measure : Subsystem
  usw_ctrl_fieldbus : Subsystem  Commented=on
  usw_fieldbus : Subsystem
  tag scope: isu_pu_dbu_fb_dbv=global, isv_pu_dbv=global, isw_pu_dbw_fb_dbv=global, motor_phase_mb_fb_dbv=global, motor_torque_ref_dbu_fb_dbv=global, usu_pu_dbu_fb_dbv=global, usv_pu_dbv=global, usw_pu_dbw_fb_dbv=global
  wires:
  motor_phase_fieldbus/1(motor_phase_fb) -> [motor_phase_mb_fb_dbv]
  [motor_phase_mb] -> motor_phase_fieldbus/1(motor_phase)
  [isw_pu_dbw] -> isw_fieldbus/1(is)
  isv_fieldbus/1(is_fb) -> [isu_pu_dbu_fb_dbv]
  isu_measure/1(is_pu) -> [isv_pu_dbv]
  [isu_pu_dbu] -> isv_fieldbus/1(is)
  [isv_dbv] -> isu_measure/1(is)
  isw_fieldbus/1(is_fb) -> [isw_pu_dbw_fb_dbv]
  [usv_dbv] -> usv_measure/1(us)
  usv_measure/1(us_pu) -> [usv_pu_dbv]
  [usw_pu_dbw] -> usw_fieldbus/1(us)
  [usu_pu_dbu] -> usu_fieldbus/1(us)
  usw_fieldbus/1(us_fb) -> [usw_pu_dbw_fb_dbv]
  usu_fieldbus/1(us_fb) -> [usu_pu_dbu_fb_dbv]
  [motor_torque_ref_dbu] -> motor_torque_fieldbus/1(us)
  motor_torque_fieldbus/1(us_fb) -> [motor_torque_ref_dbu_fb_dbv]
  From8/1 -> usw_ctrl_fieldbus/1(u_ctrl)
  usw_ctrl_fieldbus/1(u_ctrl_fb) -> Goto9/1
  usu_ctrl_fieldbus/1(u_ctrl_fb) -> Goto8/1
  From7/1 -> usu_ctrl_fieldbus/1(u_ctrl)

== system afe_rst_inv_psm_distributed_control_two_delays/INV-Modular/inv_leg_v/modulator/sv_pwm ==
  ab : Inport
  enable : Inport  Port=2
  Bus Selector : BusSelector  OutputSignals=db
  Bus Selector1 : BusSelector  OutputSignals=motor_ualpha_ctrl,motor_ubeta_ctrl
  C Caller : CCaller  FunctionName=sv_pwm_process_simulink  PortSpecificationStruct="%)30     .    N @   8    (     @         %    \"     4    !     0         %  0 \"0    $    _    07)G3F%M90  4&]R=$YA;64 4V-O<&4     26YD97@     5'EP90      4VEZ90      27-';&]B86P   X    P    !@    @    $          4    (     0    ,    !         !   P!O=70 #@   #     &    \"     0         !0    @    !     P    $         $  # &]U=  .    .     8    (    !          %    \"     $    &     0         0   ...(+2630 chars)"  SampleTime=ts_inv
  Constant : Constant  Value=ts_inv
  Data Type Conversion1 : DataTypeConversion  OutDataTypeStr=double  SaturateOnIntegerOverflow=off  RndMeth=Floor
  Data Type Conversion15 : DataTypeConversion  OutDataTypeStr=single  SaturateOnIntegerOverflow=off  RndMeth=Floor
  Data Type Conversion16 : DataTypeConversion  OutDataTypeStr=single  SaturateOnIntegerOverflow=off  RndMeth=Floor
  Data Type Conversion17 : DataTypeConversion  OutDataTypeStr=uint32  SaturateOnIntegerOverflow=off  RndMeth=Floor
  Data Type Conversion18 : DataTypeConversion  OutDataTypeStr=single  SaturateOnIntegerOverflow=off  RndMeth=Floor
  Zero-Order Hold{,1..3} (4 alike) : ZeroOrderHold  SampleTime=ts_afe
  modulator : Subsystem
  firing_gates : Outport
  wires:
  Bus Selector/1 -> Data Type Conversion1/1  "<db>"
  Zero-Order Hold/1 -> C Caller/1
  Zero-Order Hold2/1 -> C Caller/3
  Constant/1 -> Data Type Conversion16/1
  Data Type Conversion18/1 -> Zero-Order Hold/1
  enable/1 -> Data Type Conversion17/1
  Data Type Conversion16/1 -> Zero-Order Hold2/1
  Zero-Order Hold1/1 -> C Caller/2
  Data Type Conversion17/1 -> Zero-Order Hold3/1
  Zero-Order Hold3/1 -> C Caller/4
  Data Type Conversion15/1 -> Zero-Order Hold1/1
  C Caller/1 -> Bus Selector/1  "out"
  modulator/1(firing_gates) -> firing_gates/1
  ab/1 -> Bus Selector1/1
  Bus Selector1/1 -> Data Type Conversion18/1  "<motor_ualpha_ctrl>"
  Bus Selector1/2 -> Data Type Conversion15/1  "<motor_ubeta_ctrl>"
  Data Type Conversion1/1 -> modulator/1(mv)  "dv"

== system afe_rst_inv_psm_distributed_control_two_delays/INV-Modular/inv_leg_v/solid_state_inverter/switch_1 ==
  Diode : fl_lib/Electrical/Electrical Elements/Diode  Vf=Vgamma V  Ron=Ron Ohm  Goff=1e-8 1/Ohm  i_specify=off  i_priority=None  i=0 A  i_nominal_specify=off  i_nominal_value=1  i_nominal_unit=A  v_specify=off  v_priority=None  v=0 V  v_nominal_specify=off  v_nominal_value=1  v_nominal_unit=V
  Switch : fl_lib/Electrical/Electrical Elements/Switch  R_closed=Ron Ohm  G_open=1e-8 1/Ohm  Threshold=7.5  i_specify=off  i_priority=None  i=0 A  i_nominal_specify=off  i_nominal_value=1  i_nominal_unit=A  v_specify=off  v_priority=None  v=0 V  v_nominal_specify=off  v_nominal_value=1  v_nominal_unit=V
  snubber : fl_lib/Electrical/Electrical Elements/Capacitor  c=Csnubber F  r=Rsnubber Ohm  g=0 1/Ohm  i_specify=off  i_priority=None  i=0 A  i_nominal_specify=off  i_nominal_value=1  i_nominal_unit=A  v_specify=off  v_priority=None  v=0 V  v_nominal_specify=off  v_nominal_value=1  v_nominal_unit=V  vc_specify=off  vc_priority=High  vc=0 V  vc_nominal_specify=off  vc_nominal_value=1  vc_nominal_unit=V
  G : PMIOPort  Side=Left
  C : PMIOPort  Port=2  Side=Left
  E : PMIOPort  Port=3  Side=Right
  connections:
  Switch/RConn2 -- C/RConn1 -- snubber/LConn1 -- Diode/RConn1
  Switch/RConn1 -- G/RConn1
  Switch/LConn1 -- E/RConn1 -- snubber/RConn1 -- Diode/LConn1

== system afe_rst_inv_psm_distributed_control_two_delays/INV-Modular/inv_leg_v/solid_state_inverter/switch_2 ==
  Diode : fl_lib/Electrical/Electrical Elements/Diode  Vf=Vgamma V  Ron=Ron Ohm  Goff=1e-8 1/Ohm  i_specify=off  i_priority=None  i=0 A  i_nominal_specify=off  i_nominal_value=1  i_nominal_unit=A  v_specify=off  v_priority=None  v=0 V  v_nominal_specify=off  v_nominal_value=1  v_nominal_unit=V
  Switch : fl_lib/Electrical/Electrical Elements/Switch  R_closed=Ron Ohm  G_open=1e-8 1/Ohm  Threshold=7.5  i_specify=off  i_priority=None  i=0 A  i_nominal_specify=off  i_nominal_value=1  i_nominal_unit=A  v_specify=off  v_priority=None  v=0 V  v_nominal_specify=off  v_nominal_value=1  v_nominal_unit=V
  snubber : fl_lib/Electrical/Electrical Elements/Capacitor  c=Csnubber F  r=Rsnubber Ohm  g=0 1/Ohm  i_specify=off  i_priority=None  i=0 A  i_nominal_specify=off  i_nominal_value=1  i_nominal_unit=A  v_specify=off  v_priority=None  v=0 V  v_nominal_specify=off  v_nominal_value=1  v_nominal_unit=V  vc_specify=off  vc_priority=High  vc=0 V  vc_nominal_specify=off  vc_nominal_value=1  vc_nominal_unit=V
  G : PMIOPort  Side=Left
  C : PMIOPort  Port=2  Side=Left
  E : PMIOPort  Port=3  Side=Right
  connections:
  E/RConn1 -- Switch/LConn1 -- snubber/RConn1 -- Diode/LConn1
  Switch/RConn1 -- G/RConn1
  C/RConn1 -- Switch/RConn2 -- snubber/LConn1 -- Diode/RConn1
